simulink model "flcpid"  (R2026b)
settings: Solver=VariableStepAuto
settings Model: Creator=SURAJ KUMAR  LastModifiedBy=SURAJ KUMAR

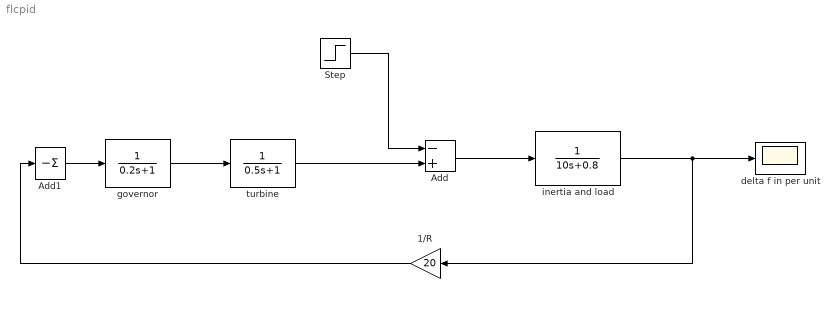
== system flcpid ==
  1/R : Gain  Gain=20
  Add : Sum  Inputs=-+
  Add1 : Sum  Inputs=-
  Step : Step  Time=100  InitialValue=0.2  FinalValue=0.2  SampleTime=0
  "delta f in per unit " : Scope
  "governor " : TransferFcn  Denominator=[0.2 1]
  "inertia and load " : TransferFcn  Denominator=[10 0.8]
  "turbine " : TransferFcn  Denominator=[0.5 1]
  wires:
  1/R/1 -> Add1/1
  Step/1 -> Add/1
  "turbine "/1 -> Add/2
  "inertia and load "/1 -> "delta f in per unit "/1, 1/R/1
  Add1/1 -> "governor "/1
  Add/1 -> "inertia and load "/1
  "governor "/1 -> "turbine "/1
